simulink model "bms"  (R2025b)
settings: configuration reference "cfgBMS" (kept outside this file)
values from neighbouring files (symbols this model uses):
  BMS_iPlausMax = 200.0    [bms.sldd]
  BMS_iRest = 0.2    [bms.sldd]
  BMS_nRetryMax = 3.0    [bms.sldd]
  BMS_ocvSoc : value not decoded    [bms.sldd]
  BMS_ocvV : value not decoded    [bms.sldd]
  BMS_Qnom = 23.45    [bms.sldd]
  BMS_soaLim : value not decoded    [bms.sldd]
  BMS_socMismatchTol = 0.1    [bms.sldd]
  BMS_tCloseMax = 0.5    [bms.sldd]
  BMS_tDiagClear = 1.0    [bms.sldd]
  BMS_tDiagSet = 0.5    [bms.sldd]
  BMS_tInitMax = 10.0    [bms.sldd]
  BMS_tInitSettle = 1.0    [bms.sldd]
  BMS_tPlausRange : value not decoded    [bms.sldd]
  BMS_tPowerPress = 1.0    [bms.sldd]
  BMS_tRecover = 5.0    [bms.sldd]
  BMS_tRelax = 7200.0    [bms.sldd]
  BMS_tResetPress = 3.0    [bms.sldd]
  BMS_tRestRecal = 600.0    [bms.sldd]
  BMS_tRetryReset = 60.0    [bms.sldd]
  BMS_Ts = 0.1    [bms.sldd]
  BMS_tStale : value not decoded    [bms.sldd]
  BMS_vPlausRange : value not decoded    [bms.sldd]
libraries: simulink x4
(part 1 of 2)
settings Model: DataDictionary=bms.sldd  Creator=SC-Br  LastModifiedBy=SC-Br
settings ConfigSetRef: SourceName=cfgBMS

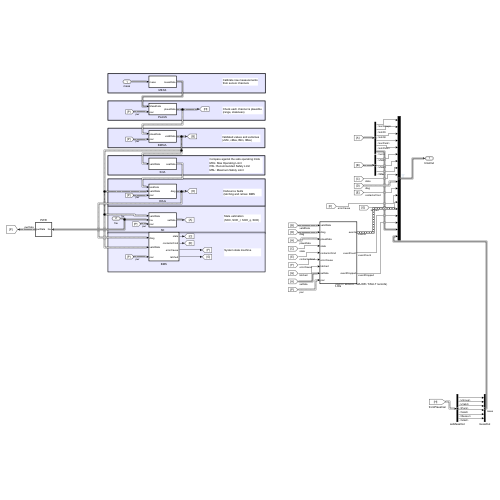
[thumbnail: Simulink's stored preview of the top-level diagram]
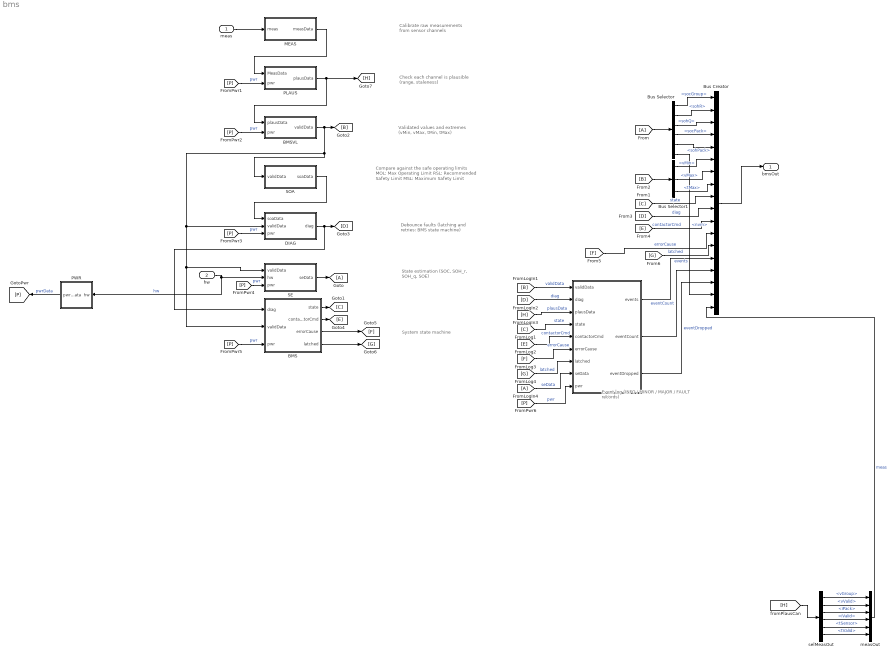
== system bms ==
  note: Calibrate raw measurements
      | from sensor channels
  note: Check each channel is plausible
      | (range, staleness)
  note: Validated values and extremes
      | (vMin, vMax, tMin, tMax)
  note: Compare against the safe operating limits
      | MOL: Max Operating Limit
      | RSL: Recommended Safety Limit
      | MSL: Maximum Safety Limit
  note: Debounce faults
      | (latching and retries: BMS state machine)
  note: State estimation
      | (SOC, SOH_r, SOH_q, SOE)
  note: System state machine
  note: Event log
      | (INFO / MINOR / MAJOR / FAULT records)
  meas : Inport  OutDataTypeStr=Bus: SENS_measBus  SampleTime=BMS_Ts
  hw : Inport  Port=2  OutDataTypeStr=Bus: BMS_hwIn  SampleTime=BMS_Ts
  BMS : Subsystem  TreatAsAtomicUnit=on  RTWFcnName=BMS_Step
      settings: RTWSystemCode=Nonreusable function  RTWFcnNameOpts=User specified  RTWFileNameOpts=Use function name
  BMSVL : Subsystem  TreatAsAtomicUnit=on  RTWFcnName=BMSVL_Step
      settings: RTWSystemCode=Nonreusable function  RTWFcnNameOpts=User specified  RTWFileNameOpts=Use function name
  Bus Creator : BusCreator  Inputs=18  NonVirtualBus=on
  Bus Selector : BusSelector  OutputSignals=socGroup,sohR,sohQ,socPack,sohPack,nvm
  Bus Selector1 : BusSelector  OutputSignals=vMin,vMax,tMax
  DIAG : Subsystem  TreatAsAtomicUnit=on  RTWFcnName=DIAG_Step
      settings: RTWSystemCode=Nonreusable function  RTWFcnNameOpts=User specified  RTWFileNameOpts=Use function name
  From : From
  FromLogIn4 : From
  Goto : Goto
  LOG : Subsystem  TreatAsAtomicUnit=on  RTWFcnName=LOG_Step
      settings: RTWSystemCode=Nonreusable function  RTWFcnNameOpts=User specified  RTWFileNameOpts=Use function name
  MEAS : Subsystem  TreatAsAtomicUnit=on  RTWFcnName=MEAS_Step
      settings: RTWSystemCode=Nonreusable function  RTWFcnNameOpts=User specified  RTWFileNameOpts=Use function name
  PLAUS : Subsystem  TreatAsAtomicUnit=on  RTWFcnName=PLAUS_Step
      settings: RTWSystemCode=Nonreusable function  RTWFcnNameOpts=User specified  RTWFileNameOpts=Use function name
  PWR : Subsystem  TreatAsAtomicUnit=on  RTWFcnName=PWR_Step
      settings: RTWSystemCode=Nonreusable function  RTWFcnNameOpts=User specified  RTWFileNameOpts=Use function name
  SE : Subsystem  TreatAsAtomicUnit=on  RTWFcnName=SE_Step
      settings: RTWSystemCode=Nonreusable function  RTWFcnNameOpts=User specified  RTWFileNameOpts=Use function name
  SOA : Subsystem  TreatAsAtomicUnit=on  RTWFcnName=SOA_Step
      settings: RTWSystemCode=Nonreusable function  RTWFcnNameOpts=User specified  RTWFileNameOpts=Use function name
  measOut : BusCreator  Inputs=6  OutDataTypeStr=Bus: BMS_measOut
  selMeasOut : BusSelector  OutputSignals=vGroup,vValid,iPack,iValid,tSensor,tValid
  bmsOut : Outport  OutDataTypeStr=Bus: BMS_outBus  BusOutputAsStruct=on
  wires:
  meas/1 -> MEAS/1(meas)
  MEAS/1(measData) -> PLAUS/1(MeasData)
  SOA/1(soaData) -> DIAG/1(soaData)
  SE/1(seData) -> Goto/1
  BMS/1(state) -> [C]
  From/1 -> Bus Selector/1
  [B] -> Bus Selector1/1
  Bus Selector1/1 -> Bus Creator/6  "<vMin>"
  [C] -> Bus Creator/9  "state"
  BMS/2(contactorCmd) -> [E]
  [E] -> Bus Creator/11  "contactorCmd"
  Bus Selector1/3 -> Bus Creator/8  "<tMax>"
  Bus Selector1/2 -> Bus Creator/7  "<vMax>"
  Bus Selector/5 -> Bus Creator/5  "<sohPack>"
  Bus Selector/4 -> Bus Creator/4  "<socPack>"
  Bus Selector/3 -> Bus Creator/3  "<sohQ>"
  Bus Selector/2 -> Bus Creator/2  "<sohR>"
  Bus Selector/1 -> Bus Creator/1  "<socGroup>"
  [D] -> Bus Creator/10  "diag"
  Bus Creator/1 -> bmsOut/1
  DIAG/1(diag) -> [D], BMS/1(diag)
  BMSVL/1(validData) -> [B], BMS/2(validData), SE/1(validData), DIAG/2(validData), SOA/1(validData)
  [H] -> LOG/3(plausData)  "plausData"
  [D] -> LOG/2(diag)  "diag"
  [B] -> LOG/1(validData)  "validData"
  [G] -> LOG/7(latched)  "latched"
  [F] -> LOG/6(errorCause)  "errorCause"
  [E] -> LOG/5(contactorCmd)  "contactorCmd"
  [C] -> LOG/4(state)  "state"
  PLAUS/1(plausData) -> [H], BMSVL/1(plausData)
  BMS/3(errorCause) -> [F]
  [F] -> Bus Creator/12  "errorCause"
  BMS/4(latched) -> [G]
  [G] -> Bus Creator/13  "latched"
  LOG/1(events) -> Bus Creator/14  "events"
  LOG/2(eventCount) -> Bus Creator/15  "eventCount"
  LOG/3(eventDropped) -> Bus Creator/16  "eventDropped"
  Bus Selector/6 -> Bus Creator/17  "<nvm>"
  hw/1 -> PWR/1(hw), SE/2(hw)  "hw"
  FromLogIn4/1 -> LOG/8(seData)  "seData"
  PWR/1(pwrData) -> [P]  "pwrData"
  [P] -> PLAUS/2(pwr)  "pwr"
  [P] -> BMSVL/2(pwr)  "pwr"
  [P] -> DIAG/3(pwr)  "pwr"
  [P] -> SE/3(pwr)  "pwr"
  [P] -> BMS/3(pwr)  "pwr"
  [P] -> LOG/9(pwr)  "pwr"
  [H] -> selMeasOut/1
  selMeasOut/1 -> measOut/1  "<vGroup>"
  selMeasOut/2 -> measOut/2  "<vValid>"
  selMeasOut/3 -> measOut/3  "<iPack>"
  selMeasOut/4 -> measOut/4  "<iValid>"
  selMeasOut/5 -> measOut/5  "<tSensor>"
  selMeasOut/6 -> measOut/6  "<tValid>"
  measOut/1 -> Bus Creator/18  "meas"

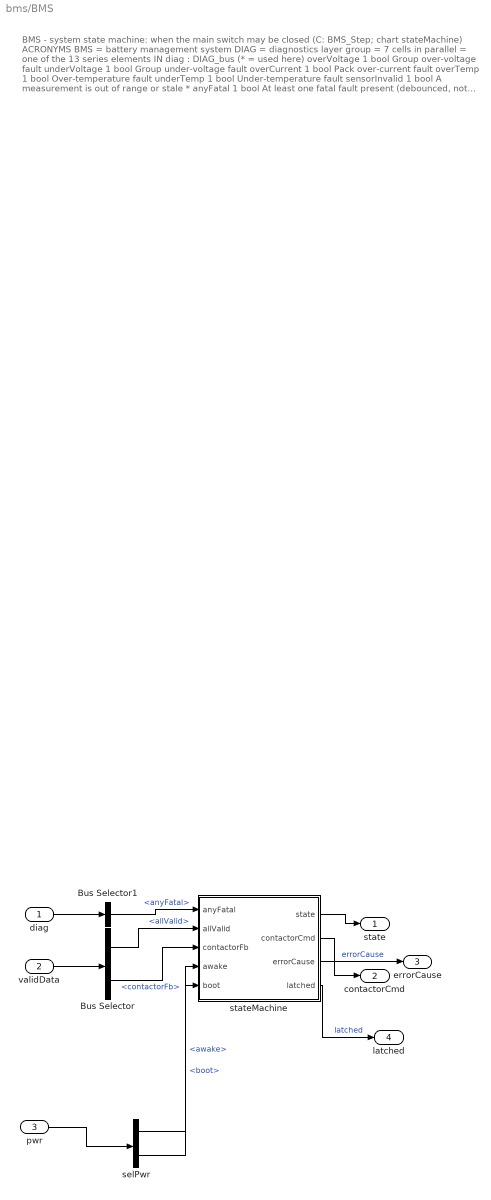
== system bms/BMS ==
  note: BMS - system state machine: when the main switch may be closed   (C: BMS_Step; chart stateMachine)
      |
      | ACRONYMS
      |   BMS = battery management system
      |   DIAG = diagnostics layer
      |   group = 7 cells in parallel = one of the 13 series elements
      |
      | IN   diag : DIAG_bus   (* = used here)
      |     overVoltage    1     bool  Group over-voltage fault
      |     underVoltage   1     bool  Group under-voltage fault
      |     overCurrent    1     bool  Pack over-current fault
      |     overTemp       1     bool  Over-temperature fault
      |     underTemp      1     bool  Under-temperature fault
      |     sensorInvalid  1     bool  A measurement is out of range or stale
      |   * anyFatal       1     bool  At least one fatal fault present (debounced, not latched: latching and retries are done by the BMS state machine)
      |     level          6x1   -     Debounced limit level per quantity [OV UV OCdchg OCchg OT UT]: 0 none, 1 MOL (MINOR), 2 RSL (MAJOR), 3 MSL (FAULT)
      |     excursion      6x1   bool  MSL exceeded but cleared before BMS_tDiagSet (one-step pulse), same order as level
      |
      | IN   validData : BMS_validData   (* = used here)
      |     vGroup         13x1  V     Validated group voltages
      |     iPack          1     A     Validated pack current
      |     tSensor        26x1  K     Validated temperatures
      |     vMin           1     V     Lowest VALID group voltage (last valid value held if none valid)
      |     vMax           1     V     Highest VALID group voltage (last valid value held if none valid)
      |     tMin           1     K     Lowest VALID temperature (last valid value held if none valid)
      |     tMax           1     K     Highest VALID temperature (last valid value held if none valid)
      |   * allValid       1     bool  Every channel plausible
      |   * contactorFb    1     bool  Validated main contactor feedback: true = closed
      |     measReady      1     bool  Every sensor type has delivered a new sample since start-up (latched)
      |     vMinIdx        1     -     Group (1-13) with the lowest valid voltage; 0 = none valid yet
      |     vMaxIdx        1     -     Group (1-13) with the highest valid voltage; 0 = none valid yet
      |     tMinIdx        1     -     Sensor (1-26) with the lowest valid temperature; 0 = none valid yet
      |     tMaxIdx        1     -     Sensor (1-26) with the highest valid temperature; 0 = none valid yet
      |
      | IN   pwr : BMS_pwrData   (* = used here)
      |   * awake          1     bool  BMS on (woken by a power long press, until the next one)
      |   * boot           1     bool  One-step pulse: every layer restarts as after a power-up (wake or reset)
      |     reset          1     bool  One-step pulse: reset long press (SOC from OCV, ERROR latch cleared)
      |     powerOn        1     bool  One-step pulse: woken by the power button
      |     powerOff       1     bool  One-step pulse: switched off by the power button
      |
      | PARAMETERS (bms.sldd)
      |   BMS_tInitSettle  = 1 s   INITIALIZATION: start-up checks must pass continuously for this long before the switch is closed
      |   BMS_tInitMax     = 10 s   INITIALIZATION: time allowed to pass the checks and close the switch before ERROR
      |   BMS_tCloseMax    = 0.5 s   Time allowed for the switch feedback to confirm closed after the close command, before ERROR
      |   BMS_tRecover     = 5 s   ERROR: fault conditions must be clear continuously for this long before a retry (back to INITIALIZATION)
      |   BMS_nRetryMax    = 3    Consecutive ERROR entries allowed before ERROR latches until power cycle
      |   BMS_tRetryReset  = 60 s   Time in NORMAL after which the retry count is reset (a later fault counts as a new first fault)
      |
      | OUT  state        (Enum: BMS_state)  OFF | INITIALIZATION = switch open, checking | NORMAL = switch closed | ERROR = fault, switch open
      | OUT  contactorCmd (boolean)          main switch command: true = close
      |
      | WHAT IT DOES
      |   - OFF (at power-up, and after a power long press): switch open, nothing else runs; ON when awake
      |   - ON: entered on wake, re-entered on reset (boot): retries and latch cleared, starts in INITIALIZATION
      |   - INITIALIZATION: switch open; when allValid, no fatal fault and feedback reads open (not welded) hold for
      |     BMS_tInitSettle, command close; NORMAL once feedback confirms within BMS_tCloseMax, else ERROR
      |   - NORMAL: a fatal fault, or the feedback opening unexpectedly -> ERROR
      |   - ERROR: switch open; retry (back to INITIALIZATION) after faults clear for BMS_tRecover;
      |     stays in ERROR after BMS_nRetryMax consecutive errors (count reset after BMS_tRetryReset in NORMAL;
      |     latch cleared by power off/on or reset)
      |
      | LIMITATIONS / LATER
      |   - ERROR reason for switch faults is not reported in diag; no precharge step
  diag : Inport  OutDataTypeStr=Bus: DIAG_bus
  validData : Inport  Port=2  OutDataTypeStr=Bus: BMS_validData
  pwr : Inport  Port=3  OutDataTypeStr=Bus: BMS_pwrData
  Bus Selector : BusSelector  OutputSignals=allValid,contactorFb
  Bus Selector1 : BusSelector  OutputSignals=anyFatal
  selPwr : BusSelector  OutputSignals=awake,boot
  stateMachine : Stateflow chart  TreatAsAtomicUnit=on
      settings: PortSchema="{\"entries\":[{\"content\":{\"sides\":[{\"content\":{\"connectorIds\":[\"In2\",\"In1\",\"In3\",\"In4\",\"In5\"]},\"type\":\"ConnectorPlacement.EquallySpacedRectSide\",\"uuid\":\"bdf09f9a-ef74-417a-a74b-8069fac80c32\"},{\"content\":{\"connectorIds\":[\"Out1\",\"Out2\",\"Out3\",\"Out4\"],\"side\":\"RIGHT\"},\"type\":\"ConnectorPlacement.EquallySpacedRectSide\",\"uuid\":\"efdc4e7f-0b2a-460f-850f-5adac2b5299f\"},{\"content\":{\"side\":\"TOP\"},\"type\":\"ConnectorPlacement.EquallySpacedRectSide\",\"uuid\":\"8f94518f-3607-4448-ad64-96b4d5c18ec7\"}]},\"type\":\"ConnectorPlacement.EquallySpacedConnector\",\"uuid\":\"d3cbdcc2-ccd9-4476-a529-a2bba1fdaf2d\"}],\"packageUris\":[\"http://schema.mathworks.com/mf0/Connector/R2020b\"],\"version\":\"1.0\"}"
  state : Outport  OutDataTypeStr=Enum: BMS_state
  contactorCmd : Outport  Port=2
  errorCause : Outport  Port=3
  latched : Outport  Port=4
  wires:
  stateMachine/1(state) -> state/1
  diag/1 -> Bus Selector1/1
  validData/1 -> Bus Selector/1
  Bus Selector/1 -> stateMachine/1(allValid)  "<allValid>"
  Bus Selector/2 -> stateMachine/3(contactorFb)  "<contactorFb>"
  Bus Selector1/1 -> stateMachine/2(anyFatal)  "<anyFatal>"
  stateMachine/2(contactorCmd) -> contactorCmd/1
  stateMachine/4(latched) -> latched/1  "latched"
  stateMachine/3(errorCause) -> errorCause/1  "errorCause"
  pwr/1 -> selPwr/1
  selPwr/1 -> stateMachine/4(awake)  "<awake>"
  selPwr/2 -> stateMachine/5(boot)  "<boot>"

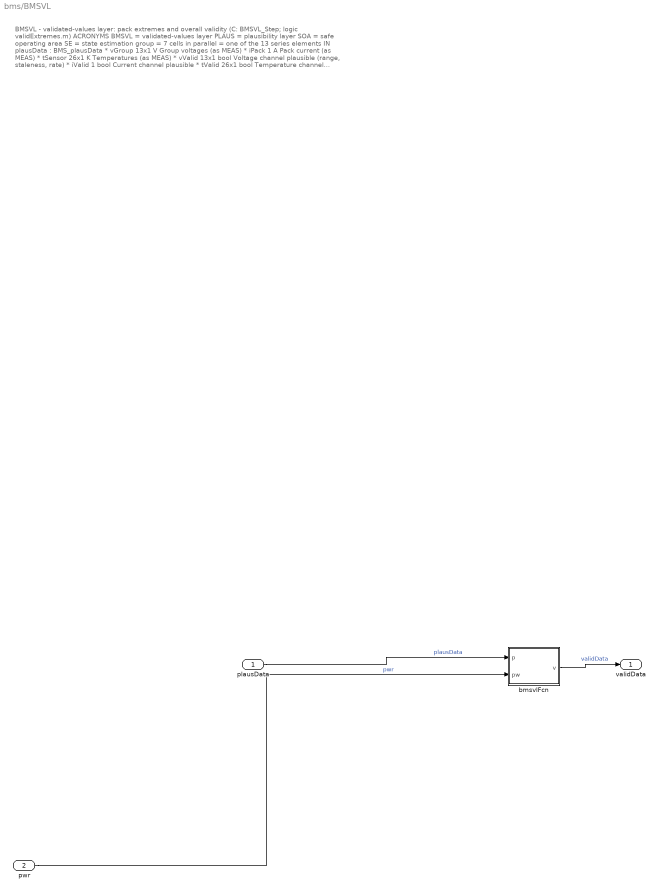
== system bms/BMSVL ==
  note: BMSVL - validated-values layer: pack extremes and overall validity   (C: BMSVL_Step; logic validExtremes.m)
      |
      | ACRONYMS
      |   BMSVL = validated-values layer
      |   PLAUS = plausibility layer
      |   SOA = safe operating area
      |   SE = state estimation
      |   group = 7 cells in parallel = one of the 13 series elements
      |
      | IN   plausData : BMS_plausData
      |   * vGroup         13x1  V     Group voltages (as MEAS)
      |   * iPack          1     A     Pack current (as MEAS)
      |   * tSensor        26x1  K     Temperatures (as MEAS)
      |   * vValid         13x1  bool  Voltage channel plausible (range, staleness, rate)
      |   * iValid         1     bool  Current channel plausible
      |   * tValid         26x1  bool  Temperature channel plausible
      |   * contactorFb    1     bool  Main contactor feedback (as MEAS)
      |   * cValid         1     bool  Contactor feedback plausible (e.g. not stale)
      |   * measReady      1     bool  Every sensor type has delivered a new sample since start-up (latched)
      |
      | IN   pwr : BMS_pwrData   (* = used here)
      |     awake          1     bool  BMS on (woken by a power long press, until the next one)
      |   * boot           1     bool  One-step pulse: every layer restarts as after a power-up (wake or reset)
      |     reset          1     bool  One-step pulse: reset long press (SOC from OCV, ERROR latch cleared)
      |     powerOn        1     bool  One-step pulse: woken by the power button
      |     powerOff       1     bool  One-step pulse: switched off by the power button
      |
      | PARAMETERS (bms.sldd)
      |   BMS_soaLim       SOA limits, each [MOL RSL MSL]: vMax vMin (V), iDchg iChg (A), tMaxDchg tMinDchg tMaxChg tMinChg (K)
      |       vMax      [4.21 4.23 4.25] V
      |       vMin      [3 2.8 2.65] V
      |       iDchg     [45 50 56] A
      |       iChg      [11.9 12.6 14] A
      |       tMaxDchg  [323.15 328.15 333.15] K  ([50 55 60] degC)
      |       tMinDchg  [273.15 268.15 263.15] K  ([0 -5 -10] degC)
      |       tMaxChg   [308.15 313.15 318.15] K  ([35 40 45] degC)
      |       tMinChg   [283.15 278.15 273.15] K  ([10 5 0] degC)
      |
      | OUT  validData : BMS_validData
      |     vGroup         13x1  V     Validated group voltages
      |     iPack          1     A     Validated pack current
      |     tSensor        26x1  K     Validated temperatures
      |     vMin           1     V     Lowest VALID group voltage (last valid value held if none valid)
      |     vMax           1     V     Highest VALID group voltage (last valid value held if none valid)
      |     tMin           1     K     Lowest VALID temperature (last valid value held if none valid)
      |     tMax           1     K     Highest VALID temperature (last valid value held if none valid)
      |     allValid       1     bool  Every channel plausible
      |     contactorFb    1     bool  Validated main contactor feedback: true = closed
      |     measReady      1     bool  Every sensor type has delivered a new sample since start-up (latched)
      |     vMinIdx        1     -     Group (1-13) with the lowest valid voltage; 0 = none valid yet
      |     vMaxIdx        1     -     Group (1-13) with the highest valid voltage; 0 = none valid yet
      |     tMinIdx        1     -     Sensor (1-26) with the lowest valid temperature; 0 = none valid yet
      |     tMaxIdx        1     -     Sensor (1-26) with the highest valid temperature; 0 = none valid yet
      |
      | WHAT IT DOES
      |   - vMin/vMax and tMin/tMax over VALID channels only: an implausible channel is reported once,
      |     as invalid, never also as an SOA limit violation
      |   - No valid channel of a type: the last valid extreme is held; before the first valid sample
      |     the extremes sit mid-way in the MOL window of BMS_soaLim (no fault: DIAG waits for measReady)
      |   - allValid = AND of every vValid, iValid, tValid and cValid; measReady passed through
      |
      | LIMITATIONS / LATER
      |   - Extremes give the worst value, not yet WHICH group or sensor (needed for fault codes)
  plausData : Inport  OutDataTypeStr=Bus: BMS_plausData
  pwr : Inport  Port=2  OutDataTypeStr=Bus: BMS_pwrData
  bmsvlFcn : MATLAB Function  TreatAsAtomicUnit=on
  validData : Outport  OutDataTypeStr=Bus: BMS_validData
  wires:
  bmsvlFcn/1(v) -> validData/1  "validData"
  plausData/1 -> bmsvlFcn/1(p)  "plausData"
  pwr/1 -> bmsvlFcn/2(pw)  "pwr"

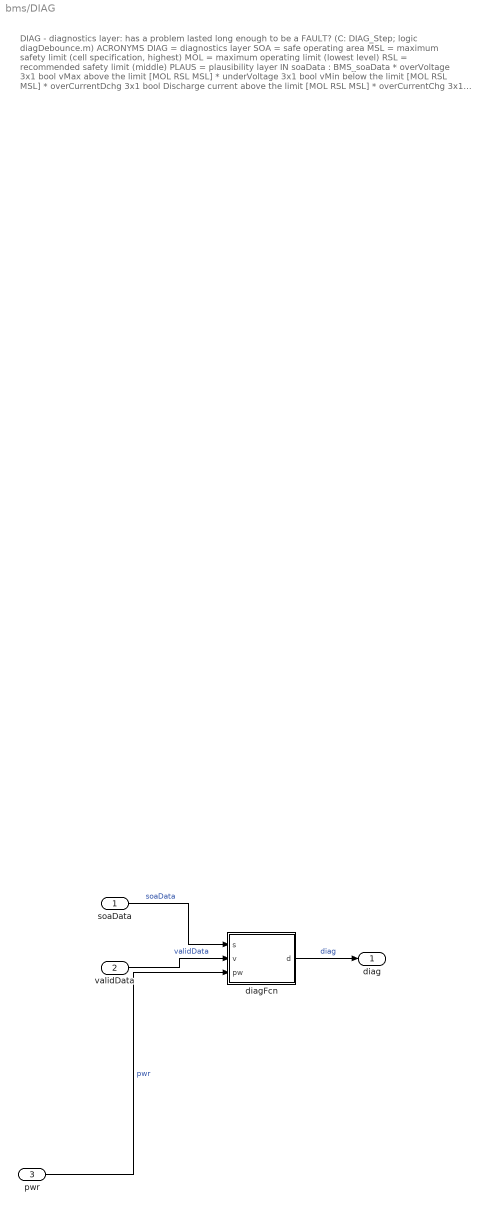
== system bms/DIAG ==
  note: DIAG - diagnostics layer: has a problem lasted long enough to be a FAULT?   (C: DIAG_Step; logic diagDebounce.m)
      |
      | ACRONYMS
      |   DIAG = diagnostics layer
      |   SOA = safe operating area
      |   MSL = maximum safety limit (cell specification, highest)
      |   MOL = maximum operating limit (lowest level)
      |   RSL = recommended safety limit (middle)
      |   PLAUS = plausibility layer
      |
      | IN   soaData : BMS_soaData
      |   * overVoltage    3x1   bool  vMax above the limit [MOL RSL MSL]
      |   * underVoltage   3x1   bool  vMin below the limit [MOL RSL MSL]
      |   * overCurrentDchg 3x1   bool  Discharge current above the limit [MOL RSL MSL]
      |   * overCurrentChg 3x1   bool  Charge current above the limit [MOL RSL MSL]
      |   * overTemp       3x1   bool  tMax above the limit [MOL RSL MSL]
      |   * underTemp      3x1   bool  tMin below the limit [MOL RSL MSL]
      |
      | IN   validData : BMS_validData   (* = used here)
      |     vGroup         13x1  V     Validated group voltages
      |     iPack          1     A     Validated pack current
      |     tSensor        26x1  K     Validated temperatures
      |     vMin           1     V     Lowest VALID group voltage (last valid value held if none valid)
      |     vMax           1     V     Highest VALID group voltage (last valid value held if none valid)
      |     tMin           1     K     Lowest VALID temperature (last valid value held if none valid)
      |     tMax           1     K     Highest VALID temperature (last valid value held if none valid)
      |   * allValid       1     bool  Every channel plausible
      |     contactorFb    1     bool  Validated main contactor feedback: true = closed
      |   * measReady      1     bool  Every sensor type has delivered a new sample since start-up (latched)
      |     vMinIdx        1     -     Group (1-13) with the lowest valid voltage; 0 = none valid yet
      |     vMaxIdx        1     -     Group (1-13) with the highest valid voltage; 0 = none valid yet
      |     tMinIdx        1     -     Sensor (1-26) with the lowest valid temperature; 0 = none valid yet
      |     tMaxIdx        1     -     Sensor (1-26) with the highest valid temperature; 0 = none valid yet
      |
      | IN   pwr : BMS_pwrData   (* = used here)
      |   * awake          1     bool  BMS on (woken by a power long press, until the next one)
      |   * boot           1     bool  One-step pulse: every layer restarts as after a power-up (wake or reset)
      |     reset          1     bool  One-step pulse: reset long press (SOC from OCV, ERROR latch cleared)
      |     powerOn        1     bool  One-step pulse: woken by the power button
      |     powerOff       1     bool  One-step pulse: switched off by the power button
      |
      | PARAMETERS (bms.sldd)
      |   BMS_tDiagSet     = 0.5 s   A limit violation or implausible measurement must persist this long to set its fault
      |   BMS_tDiagClear   = 1 s   A fault clears after its violation has been absent this long
      |   BMS_Ts           = 0.1 s   BMS task period: the rate at which the BMS reads its inputs and runs MEAS..BMS (must be a multiple of the 10 ms base rate in cfgBMS)
      |
      | OUT  diag : DIAG_bus
      |     overVoltage    1     bool  Group over-voltage fault
      |     underVoltage   1     bool  Group under-voltage fault
      |     overCurrent    1     bool  Pack over-current fault
      |     overTemp       1     bool  Over-temperature fault
      |     underTemp      1     bool  Under-temperature fault
      |     sensorInvalid  1     bool  A measurement is out of range or stale
      |     anyFatal       1     bool  At least one fatal fault present (debounced, not latched: latching and retries are done by the BMS state machine)
      |     level          6x1   -     Debounced limit level per quantity [OV UV OCdchg OCchg OT UT]: 0 none, 1 MOL (MINOR), 2 RSL (MAJOR), 3 MSL (FAULT)
      |     excursion      6x1   bool  MSL exceeded but cleared before BMS_tDiagSet (one-step pulse), same order as level
      |
      | WHAT IT DOES
      |   - Nothing is evaluated until measReady (every sensor type has delivered its first sample)
      |   - Fatal conditions: any MSL exceeded (from SOA) or any measurement implausible (allValid false)
      |   - A fault SETS once its condition has persisted BMS_tDiagSet; CLEARS once absent for BMS_tDiagClear
      |   - Debounced, not latched: remembering faults, retries and latching are in the BMS state machine
      |
      | LIMITATIONS / LATER
      |   - MOL and RSL are not used yet (future warnings and current derating)
      |   - Switch faults (stuck open, welded) are found by the state machine and are not reported here
  soaData : Inport  OutDataTypeStr=Bus: BMS_soaData
  validData : Inport  Port=2  OutDataTypeStr=Bus: BMS_validData
  pwr : Inport  Port=3  OutDataTypeStr=Bus: BMS_pwrData
  diagFcn : MATLAB Function  TreatAsAtomicUnit=on
  diag : Outport  OutDataTypeStr=Bus: DIAG_bus
  wires:
  diagFcn/1(d) -> diag/1  "diag"
  validData/1 -> diagFcn/2(v)  "validData"
  soaData/1 -> diagFcn/1(s)  "soaData"
  pwr/1 -> diagFcn/3(pw)  "pwr"

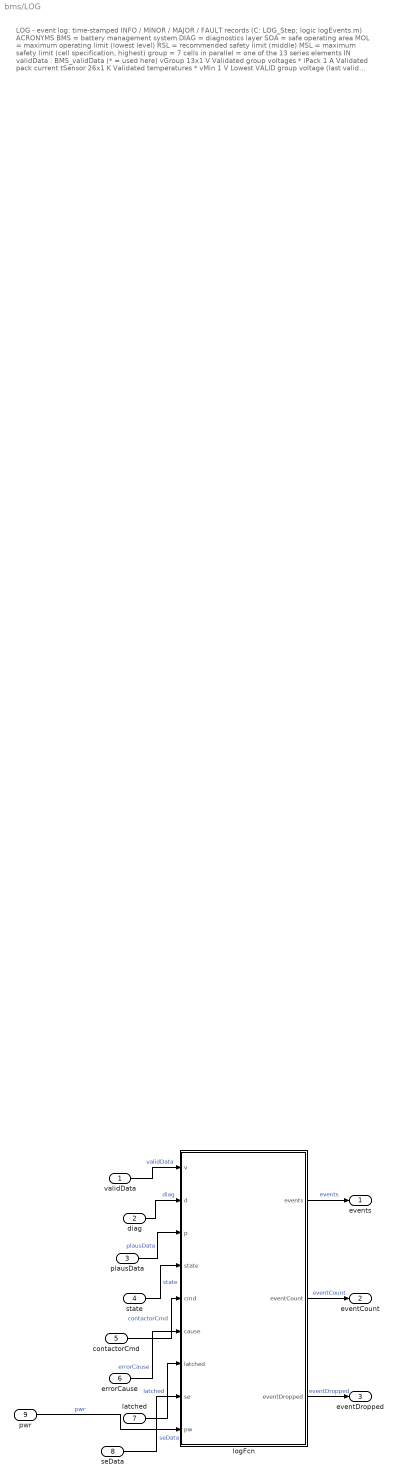
== system bms/LOG ==
  note: LOG - event log: time-stamped INFO / MINOR / MAJOR / FAULT records   (C: LOG_Step; logic logEvents.m)
      |
      | ACRONYMS
      |   BMS = battery management system
      |   DIAG = diagnostics layer
      |   SOA = safe operating area
      |   MOL = maximum operating limit (lowest level)
      |   RSL = recommended safety limit (middle)
      |   MSL = maximum safety limit (cell specification, highest)
      |   group = 7 cells in parallel = one of the 13 series elements
      |
      | IN   validData : BMS_validData   (* = used here)
      |     vGroup         13x1  V     Validated group voltages
      |   * iPack          1     A     Validated pack current
      |     tSensor        26x1  K     Validated temperatures
      |   * vMin           1     V     Lowest VALID group voltage (last valid value held if none valid)
      |   * vMax           1     V     Highest VALID group voltage (last valid value held if none valid)
      |   * tMin           1     K     Lowest VALID temperature (last valid value held if none valid)
      |   * tMax           1     K     Highest VALID temperature (last valid value held if none valid)
      |     allValid       1     bool  Every channel plausible
      |     contactorFb    1     bool  Validated main contactor feedback: true = closed
      |   * measReady      1     bool  Every sensor type has delivered a new sample since start-up (latched)
      |   * vMinIdx        1     -     Group (1-13) with the lowest valid voltage; 0 = none valid yet
      |   * vMaxIdx        1     -     Group (1-13) with the highest valid voltage; 0 = none valid yet
      |   * tMinIdx        1     -     Sensor (1-26) with the lowest valid temperature; 0 = none valid yet
      |   * tMaxIdx        1     -     Sensor (1-26) with the highest valid temperature; 0 = none valid yet
      |
      | IN   diag : DIAG_bus   (* = used here)
      |     overVoltage    1     bool  Group over-voltage fault
      |     underVoltage   1     bool  Group under-voltage fault
      |     overCurrent    1     bool  Pack over-current fault
      |     overTemp       1     bool  Over-temperature fault
      |     underTemp      1     bool  Under-temperature fault
      |   * sensorInvalid  1     bool  A measurement is out of range or stale
      |     anyFatal       1     bool  At least one fatal fault present (debounced, not latched: latching and retries are done by the BMS state machine)
      |   * level          6x1   -     Debounced limit level per quantity [OV UV OCdchg OCchg OT UT]: 0 none, 1 MOL (MINOR), 2 RSL (MAJOR), 3 MSL (FAULT)
      |   * excursion      6x1   bool  MSL exceeded but cleared before BMS_tDiagSet (one-step pulse), same order as level
      |
      | IN   plausData : BMS_plausData   (* = used here)
      |     vGroup         13x1  V     Group voltages (as MEAS)
      |     iPack          1     A     Pack current (as MEAS)
      |     tSensor        26x1  K     Temperatures (as MEAS)
      |   * vValid         13x1  bool  Voltage channel plausible (range, staleness, rate)
      |   * iValid         1     bool  Current channel plausible
      |   * tValid         26x1  bool  Temperature channel plausible
      |     contactorFb    1     bool  Main contactor feedback (as MEAS)
      |   * cValid         1     bool  Contactor feedback plausible (e.g. not stale)
      |     measReady      1     bool  Every sensor type has delivered a new sample since start-up (latched)
      |
      | IN   seData : BMS_seData   (* = used here)
      |     socGroup       13x1  1     Estimated group SOC, 0-1
      |     sohR           13x1  1     Resistance SOH per group (1 = new)
      |     sohQ           13x1  1     Capacity SOH per group (1 = new)
      |   * socPack        1     1     Pack SOC (minimum group SOC)
      |     sohPack        1     1     Pack SOH (worst group)
      |   * socInitMethod  1     -     How SOC was initialised: 0 not yet, 1 stored, 3 OCV (2 not used)
      |   * socInitMismatch 1     bool  Stored SOC disagreed with OCV beyond BMS_socMismatchTol (OCV used)
      |   * socInitDiff    1     1     Largest |stored - OCV| SOC difference over the groups at initialisation
      |   * socInitDiffIdx 1     -     Group (1-13) with that largest difference; 0 = not evaluated
      |   * socInitRest    1     s     Rest time since the stored record was saved (rtcNow - tSave); -1 = no stored record used (none valid, or reset)
      |   * socRecal       1     bool  SOC being recalibrated from OCV: pack at rest (|iPack| < BMS_iRest) for BMS_tRestRecal
      |     nvm            1     -     Record to save (current SOC, time, valid once SOC is initialised)
      |
      | IN   pwr : BMS_pwrData
      |   * awake          1     bool  BMS on (woken by a power long press, until the next one)
      |   * boot           1     bool  One-step pulse: every layer restarts as after a power-up (wake or reset)
      |   * reset          1     bool  One-step pulse: reset long press (SOC from OCV, ERROR latch cleared)
      |   * powerOn        1     bool  One-step pulse: woken by the power button
      |   * powerOff       1     bool  One-step pulse: switched off by the power button
      |
      | PARAMETERS (bms.sldd)
      |   BMS_soaLim       SOA limits, each [MOL RSL MSL]: vMax vMin (V), iDchg iChg (A), tMaxDchg tMinDchg tMaxChg tMinChg (K)
      |       vMax      [4.21 4.23 4.25] V
      |       vMin      [3 2.8 2.65] V
      |       iDchg     [45 50 56] A
      |       iChg      [11.9 12.6 14] A
      |       tMaxDchg  [323.15 328.15 333.15] K  ([50 55 60] degC)
      |       tMinDchg  [273.15 268.15 263.15] K  ([0 -5 -10] degC)
      |       tMaxChg   [308.15 313.15 318.15] K  ([35 40 45] degC)
      |       tMinChg   [283.15 278.15 273.15] K  ([10 5 0] degC)
      |   BMS_iRest        = 0.2 A   Current magnitude below which the pack is at rest: no charge temperature window (SOA), rest timer for SOC recalibration (SE) (foxBMS default 200 mA)
      |   BMS_socMismatchTol = 0.1 1   Largest stored-vs-OCV SOC difference explained by OCV error; beyond it the battery is taken as recharged or swapped while off and OCV is used
      |   BMS_Ts           = 0.1 s   BMS task period: the rate at which the BMS reads its inputs and runs MEAS..BMS (must be a multiple of the 10 ms base rate in cfgBMS)
      |
      | OUT  events : BMS_event
      |     t              1     s     BMS time since start-up (task count x BMS_Ts)
      |     severity       1     -     INFO, MINOR, MAJOR or FAULT (NONE = empty slot)
      |     code           1     -     What the record is about
      |     active         1     bool  true = raised / occurred, false = cleared
      |     location       1     -     Group 1-13 (voltage), sensor 1-26 (temperature), attempt number, new state; 0 = pack / several / n.a.
      |     level          1     -     Limit level: 1 MOL, 2 RSL, 3 MSL; 0 = not a limit record
      |     value          1     -     Measured value (V, A or K), or previous state for STATE_CHANGE
      |     limit          1     -     Limit crossed (V, A or K); 0 if not a limit record
      |     state          1     -     BMS state when recorded
      |
      | IN   state (BMS_state), contactorCmd (bool), errorCause (BMS_eventCode), latched (bool)  from the state machine
      | OUT  events = 6 slots of BMS_event per step, most severe first (severity NONE = empty slot)
      | OUT  eventCount (uint32) records since start-up | eventDropped (uint32) records lost: >6 in one step
      |
      | WHAT IT DOES
      |   - INFO: every state change, start-up check begun (attempt n) / passed, switch closed, first full sample set,
      |     SOC initialised (method, rest time); MINOR: stored SOC disagreed with OCV (recharged / swapped while off)
      |   - MINOR / MAJOR / FAULT: a quantity's debounced level rose past MOL / RSL / MSL; record again when it falls
      |     location = worst group (voltage) or sensor (temperature), value = that reading, limit = the limit crossed
      |   - MAJOR: MSL excursion (exceeded, but shorter than BMS_tDiagSet)
      |   - FAULT: sensor type invalid (location = channel, 0 = several); ERROR cause; RETRY_LIMIT when latched
      |   - A 'cleared' record keeps the severity of what cleared, with active = false
      |
      | LIMITATIONS / LATER
      |   - Records leave the BMS on BMS_outBus only (Pi bring-up: printed to the console)
      |   - Time is BMS run time (task count x BMS_Ts), not wall-clock time
  validData : Inport  OutDataTypeStr=Bus: BMS_validData
  diag : Inport  Port=2  OutDataTypeStr=Bus: DIAG_bus
  plausData : Inport  Port=3  OutDataTypeStr=Bus: BMS_plausData
  state : Inport  Port=4  OutDataTypeStr=Enum: BMS_state
  contactorCmd : Inport  Port=5  OutDataTypeStr=boolean
  errorCause : Inport  Port=6  OutDataTypeStr=Enum: BMS_eventCode
  latched : Inport  Port=7  OutDataTypeStr=boolean
  seData : Inport  Port=8  OutDataTypeStr=Bus: BMS_seData
  pwr : Inport  Port=9  OutDataTypeStr=Bus: BMS_pwrData
  logFcn : MATLAB Function  TreatAsAtomicUnit=on
  events : Outport
  eventCount : Outport  Port=2
  eventDropped : Outport  Port=3
  wires:
  logFcn/3(eventDropped) -> eventDropped/1  "eventDropped"
  logFcn/2(eventCount) -> eventCount/1  "eventCount"
  logFcn/1(events) -> events/1  "events"
  latched/1 -> logFcn/7(latched)  "latched"
  errorCause/1 -> logFcn/6(cause)  "errorCause"
  contactorCmd/1 -> logFcn/5(cmd)  "contactorCmd"
  state/1 -> logFcn/4(state)  "state"
  plausData/1 -> logFcn/3(p)  "plausData"
  diag/1 -> logFcn/2(d)  "diag"
  validData/1 -> logFcn/1(v)  "validData"
  seData/1 -> logFcn/8(se)  "seData"
  pwr/1 -> logFcn/9(pw)  "pwr"

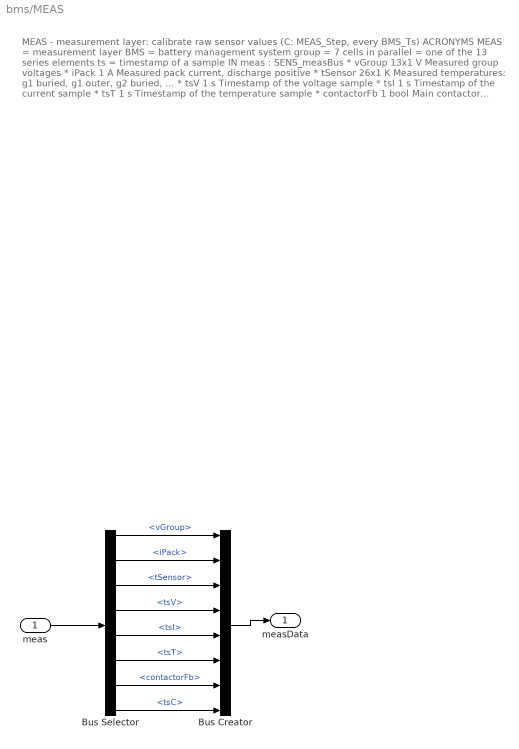
== system bms/MEAS ==
  note: MEAS - measurement layer: calibrate raw sensor values   (C: MEAS_Step, every BMS_Ts)
      |
      | ACRONYMS
      |   MEAS = measurement layer
      |   BMS = battery management system
      |   group = 7 cells in parallel = one of the 13 series elements
      |   ts = timestamp of a sample
      |
      | IN   meas : SENS_measBus
      |   * vGroup         13x1  V     Measured group voltages
      |   * iPack          1     A     Measured pack current, discharge positive
      |   * tSensor        26x1  K     Measured temperatures: g1 buried, g1 outer, g2 buried, ...
      |   * tsV            1     s     Timestamp of the voltage sample
      |   * tsI            1     s     Timestamp of the current sample
      |   * tsT            1     s     Timestamp of the temperature sample
      |   * contactorFb    1     bool  Main contactor auxiliary contact: true = closed
      |   * tsC            1     s     Timestamp of the contactor feedback sample
      |
      | OUT  measData : BMS_measData
      |     vGroup         13x1  V     Calibrated group voltages
      |     iPack          1     A     Calibrated pack current, discharge positive
      |     tSensor        26x1  K     Calibrated temperatures
      |     tsV            1     s     Timestamp of the voltage sample
      |     tsI            1     s     Timestamp of the current sample
      |     tsT            1     s     Timestamp of the temperature sample
      |     contactorFb    1     bool  Main contactor feedback: true = closed
      |     tsC            1     s     Timestamp of the contactor feedback sample
      |
      | WHAT IT DOES
      |   - Copies every measurement and its timestamp into the BMS's own bus
      |
      | LIMITATIONS / LATER
      |   - No calibration yet: later stored gain/offset per channel and current re-zero while the switch is open
  meas : Inport  OutDataTypeStr=Bus: SENS_measBus
  Bus Creator : BusCreator  Inputs=8  OutDataTypeStr=Bus: BMS_measData
  Bus Selector : BusSelector  OutputSignals=vGroup,iPack,tSensor,tsV,tsI,tsT,contactorFb,tsC
  measData : Outport  OutDataTypeStr=Bus: BMS_measData
  wires:
  meas/1 -> Bus Selector/1
  Bus Selector/1 -> Bus Creator/1  "<vGroup>"
  Bus Selector/2 -> Bus Creator/2  "<iPack>"
  Bus Selector/3 -> Bus Creator/3  "<tSensor>"
  Bus Selector/4 -> Bus Creator/4  "<tsV>"
  Bus Selector/5 -> Bus Creator/5  "<tsI>"
  Bus Selector/6 -> Bus Creator/6  "<tsT>"
  Bus Creator/1 -> measData/1
  Bus Selector/7 -> Bus Creator/7  "<contactorFb>"
  Bus Selector/8 -> Bus Creator/8  "<tsC>"

== system bms/PLAUS ==
  note: PLAUS - plausibility layer: is each sensor channel believable?   (C: PLAUS_Step; logic plausCheck.m)
      |
      | ACRONYMS
      |   PLAUS = plausibility layer
      |   SOA = safe operating area
      |   DIAG = diagnostics layer
      |   ts = timestamp of a sample
      |   V/I/T/C = voltage/current/temperature/contactor (main switch)
      |
      | IN   measData : BMS_measData
      |   * vGroup         13x1  V     Calibrated group voltages
      |   * iPack          1     A     Calibrated pack current, discharge positive
      |   * tSensor        26x1  K     Calibrated temperatures
      |   * tsV            1     s     Timestamp of the voltage sample
      |   * tsI            1     s     Timestamp of the current sample
      |   * tsT            1     s     Timestamp of the temperature sample
      |   * contactorFb    1     bool  Main contactor feedback: true = closed
      |   * tsC            1     s     Timestamp of the contactor feedback sample
      |
      | IN   pwr : BMS_pwrData   (* = used here)
      |     awake          1     bool  BMS on (woken by a power long press, until the next one)
      |   * boot           1     bool  One-step pulse: every layer restarts as after a power-up (wake or reset)
      |     reset          1     bool  One-step pulse: reset long press (SOC from OCV, ERROR latch cleared)
      |     powerOn        1     bool  One-step pulse: woken by the power button
      |     powerOff       1     bool  One-step pulse: switched off by the power button
      |
      | PARAMETERS (bms.sldd)
      |   BMS_vPlausRange  = [1 4.5] V   Plausible group-voltage range [min max]; outside = sensor fault (cell limits are SOA's)
      |   BMS_iPlausMax    = 200 A   Largest plausible |pack current| (current-sensor range)
      |   BMS_tPlausRange  = [233.15 373.15] K   Plausible temperature range [min max] (-40 to 100 degC)
      |   BMS_tStale       = [0.3 0.3 3 0.3] s   Longest time each timestamp [V I T C] may stay unchanged before the channel is stale (3 x the hardware sample period: 0.1, 0.1, 1.0, 0.1 s)
      |   BMS_Ts           = 0.1 s   BMS task period: the rate at which the BMS reads its inputs and runs MEAS..BMS (must be a multiple of the 10 ms base rate in cfgBMS)
      |
      | OUT  plausData : BMS_plausData
      |     vGroup         13x1  V     Group voltages (as MEAS)
      |     iPack          1     A     Pack current (as MEAS)
      |     tSensor        26x1  K     Temperatures (as MEAS)
      |     vValid         13x1  bool  Voltage channel plausible (range, staleness, rate)
      |     iValid         1     bool  Current channel plausible
      |     tValid         26x1  bool  Temperature channel plausible
      |     contactorFb    1     bool  Main contactor feedback (as MEAS)
      |     cValid         1     bool  Contactor feedback plausible (e.g. not stale)
      |     measReady      1     bool  Every sensor type has delivered a new sample since start-up (latched)
      |
      | WHAT IT DOES
      |   - Channel valid = first sample received AND value inside its plausible SENSOR range
      |     AND timestamp advanced within BMS_tStale
      |   - Start-up: a sensor type is invalid until its FIRST new sample (timestamp change); values before
      |     that are power-up contents. measReady latches true once all four types (V/I/T/C) have delivered
      |   - Detects sensor and wiring faults only; cell limits are checked in SOA
      |   - Reports each step as seen, no time filter (DIAG debounces)
      |
      | LIMITATIONS / LATER
      |   - One timestamp per sensor type: staleness applies to all 13 voltages (or all 26 temperatures) together
      |   - No rate-of-change check
  MeasData : Inport  OutDataTypeStr=Bus: BMS_measData
  pwr : Inport  Port=2  OutDataTypeStr=Bus: BMS_pwrData
  plausFcn : MATLAB Function  TreatAsAtomicUnit=on
  plausData : Outport  OutDataTypeStr=Bus: BMS_plausData
  wires:
  plausFcn/1(p) -> plausData/1  "plausData"
  MeasData/1 -> plausFcn/1(m)  "measData"
  pwr/1 -> plausFcn/2(pw)  "pwr"

== system bms/PWR ==
  note: PWR - power and reset buttons (long presses)   (C: PWR_Step; logic pwrManager.m)
      |
      | ACRONYMS
      |   BMS = battery management system
      |   RTC = real-time clock (battery-backed)
      |   NVM = non-volatile memory (kept over a power cycle)
      |
      | IN   hw : BMS_hwIn   (* = used here)
      |     rtcNow         1     s     Real-time clock now (battery-backed; keeps time while the BMS is off)
      |     nvm            1     -     Record read from non-volatile memory at power-up
      |   * powerBtn       1     bool  Power button pressed (long press BMS_tPowerPress: on / off)
      |   * resetBtn       1     bool  Reset button pressed (long press BMS_tResetPress: restart, SOC from OCV)
      |
      | PARAMETERS (bms.sldd)
      |   BMS_tPowerPress  = 1 s   Power button long-press time: switches the BMS on (from OFF) or off
      |   BMS_tResetPress  = 3 s   Reset button long-press time: restart with SOC from OCV, ERROR latch cleared
      |   BMS_Ts           = 0.1 s   BMS task period: the rate at which the BMS reads its inputs and runs MEAS..BMS (must be a multiple of the 10 ms base rate in cfgBMS)
      |
      | OUT  pwrData : BMS_pwrData
      |     awake          1     bool  BMS on (woken by a power long press, until the next one)
      |     boot           1     bool  One-step pulse: every layer restarts as after a power-up (wake or reset)
      |     reset          1     bool  One-step pulse: reset long press (SOC from OCV, ERROR latch cleared)
      |     powerOn        1     bool  One-step pulse: woken by the power button
      |     powerOff       1     bool  One-step pulse: switched off by the power button
      |
      | WHAT IT DOES
      |   - Starts OFF (awake = false): the switch stays open until someone switches the battery on
      |   - Power held BMS_tPowerPress: OFF -> on (awake, boot) or on -> OFF; acts once per press
      |   - Reset held BMS_tResetPress: restart (boot + reset; wakes the BMS if off): every layer restarts,
      |     SOC from OCV, ERROR latch cleared, start-up checks run again
      |
      | LIMITATIONS / LATER
      |   - Hardware: the power button drives a power latch; the BMS holds its own supply while on and
      |     releases it at switch-off (after the record is saved). Here OFF is modelled as an inactive state
  hw : Inport  OutDataTypeStr=Bus: BMS_hwIn
  pwrFcn : MATLAB Function  TreatAsAtomicUnit=on
  pwrData : Outport
  wires:
  hw/1 -> pwrFcn/1(hw)  "hw"
  pwrFcn/1(pw) -> pwrData/1  "pwrData"

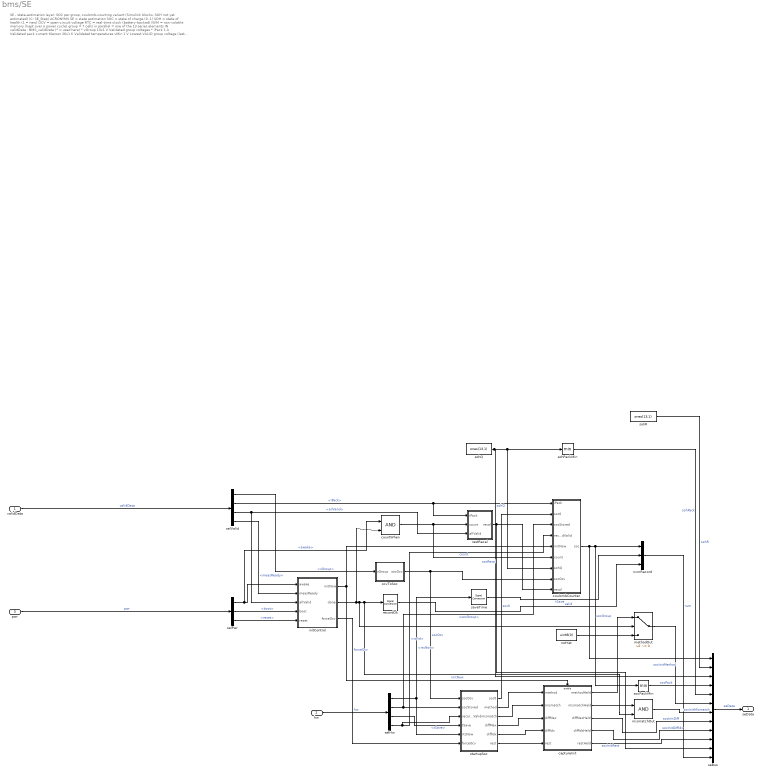
== system bms/SE ==
  note: SE - state-estimation layer: SOC per group, coulomb-counting variant (Simulink blocks; SOH not yet estimated)   (C: SE_Step)
      |
      | ACRONYMS
      |   SE = state estimation
      |   SOC = state of charge (0..1)
      |   SOH = state of health (1 = new)
      |   OCV = open-circuit voltage
      |   RTC = real-time clock (battery-backed)
      |   NVM = non-volatile memory (kept over a power cycle)
      |   group = 7 cells in parallel = one of the 13 series elements
      |
      | IN   validData : BMS_validData   (* = used here)
      |   * vGroup         13x1  V     Validated group voltages
      |   * iPack          1     A     Validated pack current
      |     tSensor        26x1  K     Validated temperatures
      |     vMin           1     V     Lowest VALID group voltage (last valid value held if none valid)
      |     vMax           1     V     Highest VALID group voltage (last valid value held if none valid)
      |     tMin           1     K     Lowest VALID temperature (last valid value held if none valid)
      |     tMax           1     K     Highest VALID temperature (last valid value held if none valid)
      |   * allValid       1     bool  Every channel plausible
      |     contactorFb    1     bool  Validated main contactor feedback: true = closed
      |   * measReady      1     bool  Every sensor type has delivered a new sample since start-up (latched)
      |     vMinIdx        1     -     Group (1-13) with the lowest valid voltage; 0 = none valid yet
      |     vMaxIdx        1     -     Group (1-13) with the highest valid voltage; 0 = none valid yet
      |     tMinIdx        1     -     Sensor (1-26) with the lowest valid temperature; 0 = none valid yet
      |     tMaxIdx        1     -     Sensor (1-26) with the highest valid temperature; 0 = none valid yet
      |
      | IN   hw : BMS_hwIn   (* = used here)
      |   * rtcNow         1     s     Real-time clock now (battery-backed; keeps time while the BMS is off)
      |   * nvm            1     -     Record read from non-volatile memory at power-up
      |     powerBtn       1     bool  Power button pressed (long press BMS_tPowerPress: on / off)
      |     resetBtn       1     bool  Reset button pressed (long press BMS_tResetPress: restart, SOC from OCV)
      |
      | IN   pwr : BMS_pwrData   (* = used here)
      |   * awake          1     bool  BMS on (woken by a power long press, until the next one)
      |   * boot           1     bool  One-step pulse: every layer restarts as after a power-up (wake or reset)
      |   * reset          1     bool  One-step pulse: reset long press (SOC from OCV, ERROR latch cleared)
      |     powerOn        1     bool  One-step pulse: woken by the power button
      |     powerOff       1     bool  One-step pulse: switched off by the power button
      |
      | PARAMETERS (bms.sldd)
      |   BMS_ocvSoc       = [0 0.1 0.2 0.3 0.4 0.5 0.6 0.7 0.8 0.9 1] 1   SOC breakpoints of the BMS OCV table (placeholder)
      |   BMS_ocvV         = [2.65 3.38 3.51 3.59 3.655 3.725 3.795 3.875 3.97 4.075 4.2] V   Cell (= group) OCV at BMS_ocvSoc, strictly increasing (placeholder)
      |   BMS_Qnom         = 23.45 A*h   Nominal (new) parallel-group capacity Q_nom: 7 cells x 3.35 Ah (placeholder). Actual capacity per group Q_act = BMS_Qnom * SOH_Q, used by coulomb counting.
      |   BMS_tRelax       = 7200 s   Rest time since switch-off after which OCV is used at start-up (cells relaxed); shorter rests keep the stored SOC (placeholder)
      |   BMS_socMismatchTol = 0.1 1   Largest stored-vs-OCV SOC difference explained by OCV error; beyond it the battery is taken as recharged or swapped while off and OCV is used
      |   BMS_iRest        = 0.2 A   Current magnitude below which the pack is at rest: no charge temperature window (SOA), rest timer for SOC recalibration (SE) (foxBMS default 200 mA)
      |   BMS_tRestRecal   = 600 s   Time at rest (|iPack| < BMS_iRest, switch closed, all valid) after which SOC is set from OCV while the rest lasts (foxBMS example: 10 min; placeholder)
      |   BMS_Ts           = 0.1 s   BMS task period: the rate at which the BMS reads its inputs and runs MEAS..BMS (must be a multiple of the 10 ms base rate in cfgBMS)
      |
      | OUT  seData : BMS_seData
      |     socGroup       13x1  1     Estimated group SOC, 0-1
      |     sohR           13x1  1     Resistance SOH per group (1 = new)
      |     sohQ           13x1  1     Capacity SOH per group (1 = new)
      |     socPack        1     1     Pack SOC (minimum group SOC)
      |     sohPack        1     1     Pack SOH (worst group)
      |     socInitMethod  1     -     How SOC was initialised: 0 not yet, 1 stored, 3 OCV (2 not used)
      |     socInitMismatch 1     bool  Stored SOC disagreed with OCV beyond BMS_socMismatchTol (OCV used)
      |     socInitDiff    1     1     Largest |stored - OCV| SOC difference over the groups at initialisation
      |     socInitDiffIdx 1     -     Group (1-13) with that largest difference; 0 = not evaluated
      |     socInitRest    1     s     Rest time since the stored record was saved (rtcNow - tSave); -1 = no stored record used (none valid, or reset)
      |     socRecal       1     bool  SOC being recalibrated from OCV: pack at rest (|iPack| < BMS_iRest) for BMS_tRestRecal
      |     nvm            1     -     Record to save (current SOC, time, valid once SOC is initialised)
      |
      | WHAT IT DOES
      |   - Blocks: ocvToSoc -> startupSoc (decision) | initControl (when) | restRecal (rest timer) | coulombCounter | captureInit (holds result)
      |   - Start-up, after every power-on or reset, on the first step with every measurement valid (switch open):
      |     socOcv = OCV-table inverse of each group voltage; rest = rtcNow - nvm.tSave
      |     record invalid or rest < 0 -> OCV | |stored - OCV| > BMS_socMismatchTol on any group
      |     (recharged or swapped while off) -> OCV, flagged | reset or rest >= BMS_tRelax -> OCV | else stored SOC
      |   - Then coulomb counting: SOC -= iPack * Ts / (3600 * BMS_Qnom * sohQ), limited to 0..1
      |   - At rest (as foxBMS): |iPack| < BMS_iRest for BMS_tRestRecal -> SOC = OCV while the rest lasts (socRecal)
      |   - socPack = lowest group SOC; nvm = record to save (valid once SOC is initialised)
      |
      | LIMITATIONS / LATER
      |   - sohR and sohQ are constant 1: NO state-of-health estimation yet (placeholders); OCV table and BMS_tRelax are placeholders
      |   - A stored-SOC error smaller than BMS_socMismatchTol is kept after a short rest; EKF / RLS variants later
      |   - At-rest OCV is the terminal voltage under the hotel load (< BMS_iRest): small IR error, as foxBMS
  validData : Inport  OutDataTypeStr=Bus: BMS_validData
  hw : Inport  Port=2  OutDataTypeStr=Bus: BMS_hwIn
  pwr : Inport  Port=3  OutDataTypeStr=Bus: BMS_pwrData
  captureInit : Subsystem
  coulombCounter : Subsystem
  countWhen : Logic  IconShape=distinctive
  initControl : Subsystem
  methodOut : Switch  Criteria=u2 ~= 0
  mismatchOut : Logic  IconShape=distinctive
  notYet : Constant  Value=uint8(0)
  nvmRecord : BusCreator  Inputs=3  OutDataTypeStr=Bus: BMS_nvmRecord
  ocvToSoc : Subsystem
  recordOk : SignalConversion  OverrideOpt=off
  restRecal : Subsystem
  saveTime : SignalConversion  OverrideOpt=off
  seBus : BusCreator  Inputs=12  OutDataTypeStr=Bus: BMS_seData
  selHw : BusSelector  OutputSignals=rtcNow,nvm.socGroup,nvm.tSave,nvm.valid
  selPwr : BusSelector  OutputSignals=awake,boot,reset
  selValid : BusSelector  OutputSignals=vGroup,iPack,allValid,measReady
  socPackMin : MinMax
  sohPackMin : MinMax
  sohQ : Constant  Value=ones(13,1)
  sohR : Constant  Value=ones(13,1)
  startupSoc : Subsystem
  seData : Outport  OutDataTypeStr=Bus: BMS_seData
  wires:
  nvmRecord/1 -> seBus/12  "nvm"
  restRecal/1(recal) -> seBus/11, coulombCounter/9(recal)  "socRecal"
  validData/1 -> selValid/1  "validData"
  hw/1 -> selHw/1  "hw"
  pwr/1 -> selPwr/1  "pwr"
  selValid/1 -> ocvToSoc/1(vGroup)  "<vGroup>"
  selPwr/1 -> initControl/1(awake), countWhen/1  "<awake>"
  selValid/4 -> initControl/2(measReady)  "<measReady>"
  selValid/3 -> restRecal/3(allValid), initControl/3(allValid)  "<allValid>"
  selPwr/2 -> initControl/4(boot)  "<boot>"
  selPwr/3 -> initControl/5(reset)  "<reset>"
  ocvToSoc/1(socOcv) -> coulombCounter/8(socOcv), startupSoc/1(socOcv)  "socOcv"
  selHw/2 -> startupSoc/2(socStored), coulombCounter/3(socStored)  "<socGroup>"
  selHw/4 -> startupSoc/3(recordValid), coulombCounter/4(recordValid)  "<valid>"
  selHw/3 -> startupSoc/4(tSave)  "<tSave>"
  selHw/1 -> startupSoc/5(rtcNow), saveTime/1  "<rtcNow>"
  initControl/3(forceOcv) -> startupSoc/6(forceOcv)  "forceOcv"
  initControl/2(done) -> mismatchOut/2, recordOk/1, methodOut/2, countWhen/2
  selValid/2 -> restRecal/1(iPack), coulombCounter/1(iPack)  "<iPack>"
  startupSoc/1(soc0) -> coulombCounter/2(soc0)  "soc0"
  initControl/1(initNow) -> coulombCounter/5(initNow), captureInit/Enable  "initNow"
  countWhen/1 -> restRecal/2(count), coulombCounter/6(count)  "count"
  sohQ/1 -> coulombCounter/7(sohQ), sohPackMin/1, seBus/3  "sohQ"
  startupSoc/2(method) -> captureInit/1(method)
  startupSoc/3(mismatch) -> captureInit/2(mismatch)
  startupSoc/4(diffMax) -> captureInit/3(diffMax)
  startupSoc/5(diffIdx) -> captureInit/4(diffIdx)
  startupSoc/6(rest) -> captureInit/5(rest)
  captureInit/1(methodHeld) -> methodOut/1
  notYet/1 -> methodOut/3
  captureInit/2(mismatchHeld) -> mismatchOut/1
  coulombCounter/1(soc) -> socPackMin/1, nvmRecord/1, seBus/1  "socGroup"
  saveTime/1 -> nvmRecord/2  "tSave"
  recordOk/1 -> nvmRecord/3  "valid"
  sohR/1 -> seBus/2  "sohR"
  socPackMin/1 -> seBus/4  "socPack"
  sohPackMin/1 -> seBus/5  "sohPack"
  methodOut/1 -> seBus/6  "socInitMethod"
  mismatchOut/1 -> seBus/7  "socInitMismatch"
  captureInit/3(diffMaxHeld) -> seBus/8  "socInitDiff"
  captureInit/4(diffIdxHeld) -> seBus/9  "socInitDiffIdx"
  captureInit/5(restHeld) -> seBus/10  "socInitRest"
  seBus/1 -> seData/1  "seData"

== system bms/SOA ==
  note: SOA - safe-operating-area layer: is any quantity beyond a limit RIGHT NOW?   (C: SOA_Step; logic soaCheck.m)
      |
      | ACRONYMS
      |   SOA = safe operating area
      |   MOL = maximum operating limit (lowest level)
      |   RSL = recommended safety limit (middle)
      |   MSL = maximum safety limit (cell specification, highest)
      |   DIAG = diagnostics layer
      |   dchg/chg = discharge/charge (current discharge-positive)
      |
      | IN   validData : BMS_validData   (* = used here)
      |     vGroup         13x1  V     Validated group voltages
      |   * iPack          1     A     Validated pack current
      |     tSensor        26x1  K     Validated temperatures
      |   * vMin           1     V     Lowest VALID group voltage (last valid value held if none valid)
      |   * vMax           1     V     Highest VALID group voltage (last valid value held if none valid)
      |   * tMin           1     K     Lowest VALID temperature (last valid value held if none valid)
      |   * tMax           1     K     Highest VALID temperature (last valid value held if none valid)
      |     allValid       1     bool  Every channel plausible
      |     contactorFb    1     bool  Validated main contactor feedback: true = closed
      |     measReady      1     bool  Every sensor type has delivered a new sample since start-up (latched)
      |     vMinIdx        1     -     Group (1-13) with the lowest valid voltage; 0 = none valid yet
      |     vMaxIdx        1     -     Group (1-13) with the highest valid voltage; 0 = none valid yet
      |     tMinIdx        1     -     Sensor (1-26) with the lowest valid temperature; 0 = none valid yet
      |     tMaxIdx        1     -     Sensor (1-26) with the highest valid temperature; 0 = none valid yet
      |
      | PARAMETERS (bms.sldd)
      |   BMS_soaLim       SOA limits, each [MOL RSL MSL]: vMax vMin (V), iDchg iChg (A), tMaxDchg tMinDchg tMaxChg tMinChg (K)
      |       vMax      [4.21 4.23 4.25] V
      |       vMin      [3 2.8 2.65] V
      |       iDchg     [45 50 56] A
      |       iChg      [11.9 12.6 14] A
      |       tMaxDchg  [323.15 328.15 333.15] K  ([50 55 60] degC)
      |       tMinDchg  [273.15 268.15 263.15] K  ([0 -5 -10] degC)
      |       tMaxChg   [308.15 313.15 318.15] K  ([35 40 45] degC)
      |       tMinChg   [283.15 278.15 273.15] K  ([10 5 0] degC)
      |   BMS_iRest        = 0.2 A   Current magnitude below which the pack is at rest: no charge temperature window (SOA), rest timer for SOC recalibration (SE) (foxBMS default 200 mA)
      |
      | OUT  soaData : BMS_soaData
      |     overVoltage    3x1   bool  vMax above the limit [MOL RSL MSL]
      |     underVoltage   3x1   bool  vMin below the limit [MOL RSL MSL]
      |     overCurrentDchg 3x1   bool  Discharge current above the limit [MOL RSL MSL]
      |     overCurrentChg 3x1   bool  Charge current above the limit [MOL RSL MSL]
      |     overTemp       3x1   bool  tMax above the limit [MOL RSL MSL]
      |     underTemp      3x1   bool  tMin below the limit [MOL RSL MSL]
      |
      | WHAT IT DOES
      |   - Compares the extremes and the current with three limits per quantity: [MOL RSL MSL]; true = exceeded
      |   - Charging (iPack < -BMS_iRest) selects the tighter charge temperature window
      |   - Instantaneous: one comparison per step, no time filter, no fault decision (that is DIAG's job)
      |
      | LIMITATIONS / LATER
      |   - MSLs from the Samsung INR18650-35E specification Ver. 1.1 x 7 cells, except the vMax MSL (4.25 V,
      |     engineering judgement: 4.20 V is the normal charge voltage); MOL and RSL margins are placeholders
  validData : Inport  OutDataTypeStr=Bus: BMS_validData
  soaFcn : MATLAB Function  TreatAsAtomicUnit=on
  soaData : Outport  OutDataTypeStr=Bus: BMS_soaData
  wires:
  soaFcn/1(s) -> soaData/1  "soaData"
  validData/1 -> soaFcn/1(v)  "validData"

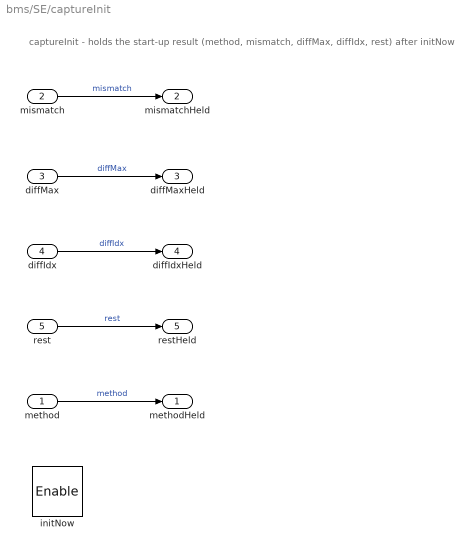
== system bms/SE/captureInit ==
  note: captureInit - holds the start-up result (method, mismatch, diffMax, diffIdx, rest) after initNow
  method : Inport
  mismatch : Inport  Port=2
  diffMax : Inport  Port=3
  diffIdx : Inport  Port=4
  rest : Inport  Port=5
  initNow : EnablePort
  methodHeld : Outport  InitialOutput=0
  mismatchHeld : Outport  Port=2  InitialOutput=0
  diffMaxHeld : Outport  Port=3  InitialOutput=0
  diffIdxHeld : Outport  Port=4  InitialOutput=0
  restHeld : Outport  Port=5  InitialOutput=0
  wires:
  rest/1 -> restHeld/1  "rest"
  diffIdx/1 -> diffIdxHeld/1  "diffIdx"
  diffMax/1 -> diffMaxHeld/1  "diffMax"
  mismatch/1 -> mismatchHeld/1  "mismatch"
  method/1 -> methodHeld/1  "method"

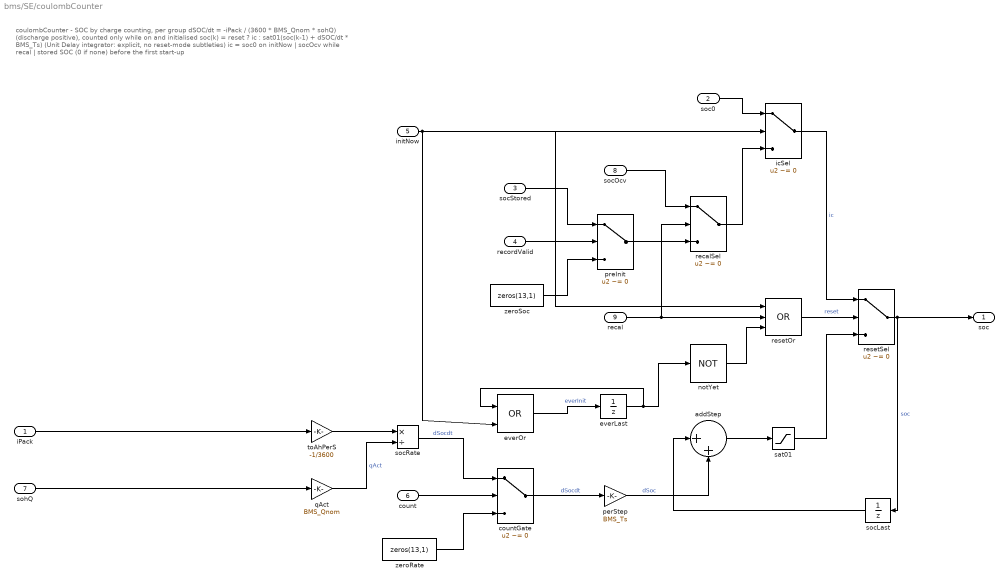
== system bms/SE/coulombCounter ==
  note: coulombCounter - SOC by charge counting, per group
      |   dSOC/dt = -iPack / (3600 * BMS_Qnom * sohQ)  (discharge positive), counted only while on and initialised
      |   soc(k) = reset ? ic : sat01(soc(k-1) + dSOC/dt * BMS_Ts)   (Unit Delay integrator: explicit, no reset-mode subtleties)
      |   ic = soc0 on initNow | socOcv while recal | stored SOC (0 if none) before the first start-up
  iPack : Inport
  soc0 : Inport  Port=2
  socStored : Inport  Port=3
  recordValid : Inport  Port=4
  initNow : Inport  Port=5
  count : Inport  Port=6
  sohQ : Inport  Port=7
  socOcv : Inport  Port=8
  recal : Inport  Port=9
  addStep : Sum  Inputs=|++
  countGate : Switch  Criteria=u2 ~= 0
  everLast : UnitDelay  InitialCondition=false  SampleTime=-1
  everOr : Logic  Operator=OR  IconShape=distinctive
  icSel : Switch  Criteria=u2 ~= 0
  notYet : Logic  Operator=NOT  IconShape=distinctive
  perStep : Gain  Gain=BMS_Ts
  preInit : Switch  Criteria=u2 ~= 0
  qAct : Gain  Gain=BMS_Qnom
  recalSel : Switch  Criteria=u2 ~= 0
  resetOr : Logic  Operator=OR  Inputs=3  IconShape=distinctive
  resetSel : Switch  Criteria=u2 ~= 0
  sat01 : Saturate  UpperLimit=1  LowerLimit=0
  socLast : UnitDelay  SampleTime=-1
  socRate : Product  Inputs=*/
  toAhPerS : Gain  Gain=-1/3600
  zeroRate : Constant  Value=zeros(13,1)
  zeroSoc : Constant  Value=zeros(13,1)
  soc : Outport
  wires:
  resetOr/1 -> resetSel/2  "reset"
  notYet/1 -> resetOr/3
  everOr/1 -> everLast/1  "everInit"
  everLast/1 -> notYet/1, everOr/1
  resetSel/1 -> socLast/1, soc/1  "soc"
  sat01/1 -> resetSel/3
  icSel/1 -> resetSel/1  "ic"
  addStep/1 -> sat01/1
  perStep/1 -> addStep/2  "dSoc"
  socLast/1 -> addStep/1
  countGate/1 -> perStep/1  "dSocdt"
  initNow/1 -> resetOr/1, everOr/2, icSel/2
  soc0/1 -> icSel/1
  zeroSoc/1 -> preInit/3
  recordValid/1 -> preInit/2
  socStored/1 -> preInit/1
  zeroRate/1 -> countGate/3
  count/1 -> countGate/2
  socRate/1 -> countGate/1  "dSocdt"
  qAct/1 -> socRate/2  "qAct"
  toAhPerS/1 -> socRate/1
  sohQ/1 -> qAct/1
  iPack/1 -> toAhPerS/1
  socOcv/1 -> recalSel/1
  recal/1 -> resetOr/2, recalSel/2
  preInit/1 -> recalSel/3
  recalSel/1 -> icSel/3
